simulink model "snap_adc5g_spec"  (R2019a)
settings: Solver=VariableStepDiscrete  StartTime=0.0  StopTime=10.0  RelTol=1e-3
undefined symbols (not defined in the file): pfb_coeff_gen_calc
libraries: xbsIndex_r4 x13965, casper_library_misc x80, casper_library_delays x43, xps_library x5, xbsReplacements_r4 x2, casper_library_communications x1
(part 1 of 152)
settings Model: Creator=jackh  LastModifiedBy=jackh
settings DataIOCC: ReturnWorkspaceOutputs=off
settings OptimizationCC: DefaultParameterBehavior=Inlined
settings DebuggingCC: ArithmeticOperatorsInVariantConditions=warning
settings SFSimCC: SimUseLocalCustomCode=off
settings RTWCC: RTWUseLocalCustomCode=off
settings CodeAppCC: StateflowObjectComments=on

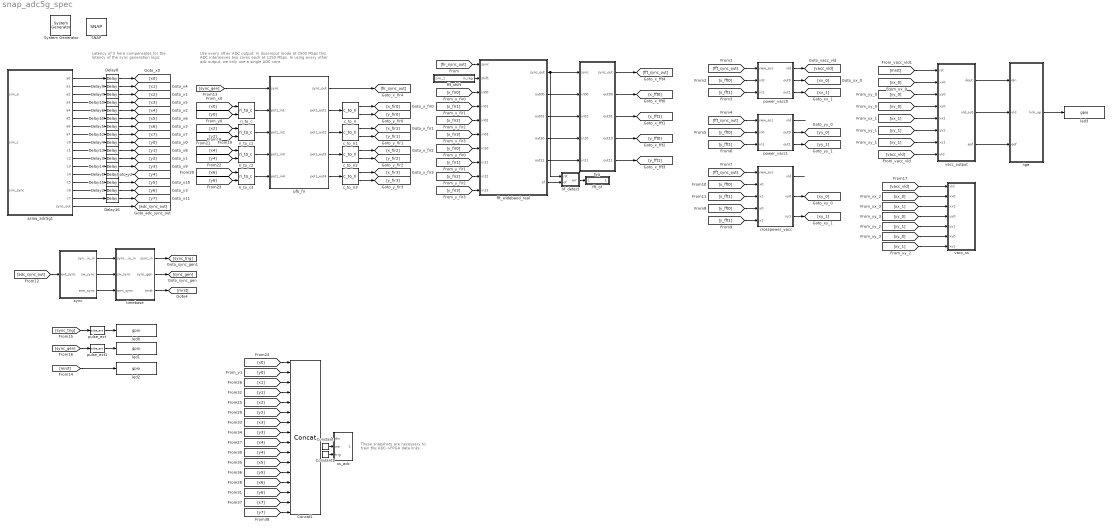
== system snap_adc5g_spec ==
  note: These snapshots are necessary
      | to train the ADC->FPGA data links.
  note: Latency of 5 here compensates
      | for the latency of the sync generation logic
  note: Use every other ADC output. In dual-input mode at 2500 MSps
      | this ADC interleaves two cores each at 1250 MSps. In using
      | every other adc output, we only use a single ADC core.
  " System Generator" : xbsIndex_r4/ System Generator  Tag=genX  xilinxfamily=kintex7  part=xc7k160t  speed=-2  package=ffg676  synthesis_tool=XST  clock_wrapper=Clock Enables  directory=/home/jackh/src/ata_snap/snap_adc5g_spec/sysgen  proj_type=Vivado  Synth_file=Vivado Synthesis Defaults  Impl_file=Vivado Implementation Defaults  testbench=off  simulink_period=1  sysclk_period=3.2  dcm_input_clock_period=10  incr_netlist=off  trim_vbits=Everywhere in SubSystem  dbl_ovrd=According to Block Masks  core_generation=According to Block Masks  run_coregen=off  deprecated_control=off  eval_field=0  block_type=sysgen
  Concat1 : xbsIndex_r4/Concat  num_inputs=16  dbl_ovrd=off  block_type=concat
  Constant : xbsIndex_r4/Constant  const=0  gui_display_data_type=Boolean  arith_type=Boolean  n_bits=16  bin_pt=14  preci_type=Single  exp_width=8  frac_width=24  explicit_period=on  period=1  equ=P=C  opselect=C  inp2=PCIN>>17  opr=+  inp1=P  carry=CIN  dbl_ovrd=off  block_type=constant
  Constant1 : xbsIndex_r4/Constant  const=0  gui_display_data_type=Boolean  arith_type=Boolean  n_bits=16  bin_pt=14  preci_type=Single  exp_width=8  frac_width=24  explicit_period=on  period=1  equ=P=C  opselect=C  inp2=PCIN>>17  opr=+  inp1=P  carry=CIN  dbl_ovrd=off  block_type=constant
  Delay{1..16} (16 alike) : xbsIndex_r4/Delay  rst=off  infoeditControl=Selection of Reset will increase slice count due to use of real FFs and instead of SRLs  en=off  latency=5  reg_retiming=off  dbl_ovrd=off  block_type=delay
      settings: block_version=11.4
  SNAP : xps_library/Platforms/SNAP  Tag=xps:xsg  hw_sys=SNAP:xc7k160t  clk_src=adc0_clk  clk_rate=1250/4  use_microblaze=on  sample_period=1  synthesis_tool=XST
      settings: SourceProductName=CASPER XPS Blockset
  asiaa_adc5g1 : Subsystem  Tag=xps:adc5g  AncestorBlock=xps_library/ADCs/asiaa_adc5g  mask(adc5g){input_mode=Two-channel -- A&C, adc_brd=ZDOK 0, demux=1:1, adc_bit_width=8, adc_clk_rate=2500, using_ctrl=on, test_ramp=off}
      mask prompts: input_mode "Input mode:"; adc_brd "ADC Board"; demux "Internal demux"; adc_bit_width "ADC Resolution (bits):"; adc_clk_rate "ADC Clock Rate (MHz):"; using_ctrl "use control"; test_ramp "start in test ramp mode"
      mask help:
      | Interface for the ASIAA 5 GSps ADC. Supports interleaving all four
      | cores using either input A or C, or interleaving two-cores each for
      | A and C. The hardware itself comes in two versions:
      |
      | DMUX 1:2 -- 4-bit samples, 4 parallel streams
      | DMUX 1:1 -- 8-bit samples, 2 parallel streams
      |
      | In either configuration this block will output 8 parallel streams
      | but the underlying interface, and the bitwidth of the samples,
      | will be different.
      mask init:
      | adc5g_init(gcb,...
      |     'input_mode', input_mode,...
      |     'demux', demux,...
      |     'adc_clk_rate', adc_clk_rate,...
      |     'adc_bit_width', adc_bit_width,...
      |     'adc_brd', adc_brd,...
      |     'using_ctrl', using_ctrl,...
      |     'test_ramp', test_ramp);
      mask TypeOptions input_mode: One-channel -- A | One-channel -- C | Two-channel -- A&C
      mask TypeOptions adc_brd: ZDOK 0 | ZDOK 1
      mask TypeOptions demux: 1:1 | 1:2
      mask Callback demux:
      | demux = get_param(gcb,'demux');
      | if(strcmp(demux,'1:1')),
      |     set_param(gcb, 'adc_bit_width', '8')
      | elseif(strcmp(demux, '1:2')),
      |     set_param(gcb, 'adc_bit_width', '4');
      | else
      | end
  c_to_ri{,1..3} (4 alike) : casper_library_misc/c_to_ri  n_bits=18  bin_pt=17
      settings: SourceProductName=CASPER DSP Blockset
  crosspower_vacc : Subsystem  mask{bw=18, nchan=2048, vacc_bw=32, vacc_bp=24}
      mask prompts: bw "Bitwidth in"; nchan "Number of channels"; vacc_bw "Vector accumulator output bitwidth"; vacc_bp "Vector accumulator output binary point"
  fft_of : Subsystem  Tag=xps:sw_reg  AncestorBlock=xps_library/Memory/software_register  mask(swreg){io_dir=To Processor, io_delay=0, init_val=0, sample_period=1, names=reg, bitwidths=1, bin_pts=0, arith_types=2, sim_port=on, show_format=on}
      mask prompts: io_dir "I/O direction"; io_delay "I/O delay"; init_val "Initial Value"; sample_period "Sample period"; names "Bitfield names [msb...lsb]"; bitwidths "Bitfield widths"; bin_pts "Bitfield binary pts"; arith_types "Bitfield types, ufix=0, fix=1, bool=2"; sim_port "Provide sim input/output?"; show_format "Print format string?"
      mask help: A 32-bit software-accessible register. Can be divided into bitfields of varying widths and types using the fields in the block mask.
      mask init:
      | swreg_init(gcb)
      settings: AttributesFormatString=1output:b = 1 bits
      mask TypeOptions io_dir: To Processor | From Processor
      mask Callback io_dir:
      | mask_enables = get_param(gcb, 'MaskEnables');
      | mask_names = get_param(gcb, 'MaskNames');
      | if strcmp(get_param(gcb, 'io_dir'), 'To Processor'),
      |     mask_enables{ismember(mask_names, 'sample_period')} = 'off';
      | else
      |     mask_enables{ismember(mask_names, 'sample_period')} = 'on';
      | end
      | set_param(gcb, 'MaskEnables', mask_enables);
      mask DialogControl ParameterTabVar0 Prompt: Setup
  fft_shift : Subsystem  Tag=xps:sw_reg  AncestorBlock=xps_library/Memory/software_register  mask(swreg){io_dir=From Processor, io_delay=0, init_val=0, sample_period=1, names=reg, bitwidths=32, bin_pts=0, arith_types=0, sim_port=on, show_format=on}
      mask prompts: io_dir "I/O direction"; io_delay "I/O delay"; init_val "Initial Value"; sample_period "Sample period"; names "Bitfield names [msb...lsb]"; bitwidths "Bitfield widths"; bin_pts "Bitfield binary pts"; arith_types "Bitfield types, ufix=0, fix=1, bool=2"; sim_port "Provide sim input/output?"; show_format "Print format string?"
      mask help: A 32-bit software-accessible register. Can be divided into bitfields of varying widths and types using the fields in the block mask.
      mask init:
      | swreg_init(gcb)
      settings: AttributesFormatString=1input:uf32.0 = 32 bits
      mask TypeOptions io_dir: To Processor | From Processor
      mask Callback io_dir:
      | mask_enables = get_param(gcb, 'MaskEnables');
      | mask_names = get_param(gcb, 'MaskNames');
      | if strcmp(get_param(gcb, 'io_dir'), 'To Processor'),
      |     mask_enables{ismember(mask_names, 'sample_period')} = 'off';
      | else
      |     mask_enables{ismember(mask_names, 'sample_period')} = 'on';
      | end
      | set_param(gcb, 'MaskEnables', mask_enables);
      mask DialogControl ParameterTabVar0 Prompt: Setup
  fft_wideband_real : Subsystem  Tag=casper:fft_wideband_real  AncestorBlock=casper_library_ffts/fft_wideband_real  mask(fft_wideband_real){n_streams=2, FFTSize=13, n_inputs=2, input_bit_width=18, bin_pt_in=17, coeff_bit_width=18, unscramble=on, async=off, floating_point=off, float_type=single, exp_width=8, frac_width=24, add_latency=1, mult_latency=2, bram_latency=3, conv_latency=1, input_latency=0, biplex_direct_latency=0, add_pipe_latency=0, mult_pipe_latency=0, quantization=Round  (unbiased: Even Values), overflow=Wrap, delays_bit_limit=8, coeffs_bit_limit=9, coeff_sharing=on, coeff_decimation=on, coeff_generation=off, cal_bits=1, n_bits_rotation=25, mult_spec=2, max_fanout=4, bitgrowth=off, max_bits=19, hardcode_shifts=off, shift_schedule=[], dsp48_adders=off}
      mask prompts: n_streams "Number simultaneous streams"; FFTSize "Size of FFT: (2^? pts)"; n_inputs "Number of Simultaneous Inputs: (2^?)"; input_bit_width "Input Bit Width"; bin_pt_in "Input binary point"; coeff_bit_width "Coefficient Bit Width"; unscramble "Unscramble output (ie, put channels in canonical order)"; async "Asynchronous operation"; floating_point "floating point"; float_type "float type"; exp_width "exponent width"; frac_width "fraction width"; add_latency "Add Latency"; mult_latency "Mult Latency"; bram_latency "BRAM Latency"; conv_latency "Convert Latency"; input_latency "Input Latency"; biplex_direct_latency "Latency between biplexes and fft_direct"; add_pipe_latency "Add Interface Pipeline Latency"; mult_pipe_latency "CMult Pipeline Latency"; quantization "Quantization Behavior"; overflow "Overflow Behavior"; delays_bit_limit "Number bits above which to store stage's delays in BRAM (2^? bits)"; coeffs_bit_limit "Number bits above which to store stage's coefficients in BRAM (2^? bits)"; coeff_sharing "BRAM sharing in coeff storage"; coeff_decimation "Store a fraction of coeff factors where useful"; coeff_generation "Generate coeffs with multipliers where useful"; cal_bits "Number calibration locations when generating coeffs (2^?)"; n_bits_rotation "Feedback rotation vector resolution"; mult_spec "Multiplier impl. (0=core, 1=embedded, 2=behavioural) (left=1st stage, or just one value)"; max_fanout "Maximum fanout"; bitgrowth "Bitgrowth instead of shifting"; max_bits "Max bits to grow to"; hardcode_shifts "Hardcode shift schedule"; shift_schedule "Shift schedule"; dsp48_adders "DSP48 adders in butterfly"
      mask help: A real-sampled wideband FFT.
      mask init:
      | fft_wideband_real_init(gcb, ...
      |     'n_streams', n_streams, ...
      |     'FFTSize', FFTSize, ...
      |     'n_inputs', n_inputs, ...
      |     'input_bit_width', input_bit_width, ...
      |     'bin_pt_in', bin_pt_in, ...
      |     'coeff_bit_width', coeff_bit_width, ...
      |     'floating_point', floating_point, ...
      |     'float_type', float_type, ...
      |     'exp_width', exp_width, ...
      |     'frac_width', frac_width, ...
      |     'unscramble', unscramble, ...
      |     'async', async, ...
      |     'add_latency', add_latency, ...
      |     'mult_latency', mult_latency, ...
      |     'bram_latency', bram_latency, ...
      |     'conv_latency', conv_latency, ...
      |     'input_latency', input_latency, ...
      |     'add_pipe_latency', add_pipe_latency, ...
      |     'mult_pipe_latency', mult_pipe_latency, ...
      |     'biplex_direct_latency', biplex_direct_latency, ...
      |     'quantization', quantization, ...
      |     'overflow', overflow, ...
      |     'delays_bit_limit', delays_bit_limit, ...
      |     'coeffs_bit_limit', coeffs_bit_limit, ...
      |     'coeff_sharing', coeff_sharing, ...
      |     'coeff_decimation', coeff_decimation, ...
      |     'coeff_generation', coeff_generation, ...
      |     'cal_bits', cal_bits, ...
      |     'n_bits_rotation', n_bits_rotation, ...
      |     'max_fanout', max_fanout, ...   
      |     'mult_spec', mult_spec, ...
      |     'bitgrowth', bitgrowth, ...
      |     'max_bits', max_bits, ...
      |     'hardcode_shifts', hardcode_shifts, ...
      |     'shift_schedule', shift_schedule, ...
      |     'dsp48_adders', dsp48_adders);
      settings: AttributesFormatString=|
      | 13 stages
      | (18,18)
      | Round  (unbiased: Even Values)
      | Wrap
      mask Help: eval('xlWeb(''http://casper.berkeley.edu/wiki/Fft_wideband_real'')')
      mask Callback floating_point:
      | onoff = get_param(gcb, 'floating_point');
      | if strcmp(onoff,'on')
      |     enable_fixpt = 'off'
      |     set_param_state(gcb, 'float_type', 'on')
      | 
      |     f_type = get_param(gcb, 'float_type')
      |     if strcmp(f_type,'custom')
      |         set_param_state(gcb, 'exp_width', 'on')
      |         set_param_state(gcb, 'frac_width', 'on')
      |     else
      |         set_param_state(gcb, 'exp_width', 'off')
      |         set_param_state(gcb, 'frac_width', 'off')
      |     end
      | 
      | 
      | else
      |     enable_fixpt = 'on'
      |     set_param_state(gcb, 'float_type', 'off')
      |     set_param_state(gcb, 'exp_width', 'off')
      |     set_param_state(gcb, 'frac_width', 'off')
      | end
      | 
      | set_param_state(gcb, 'input_bit_width', enable_fixpt)
      | set_param_state(gcb, 'bin_pt_in', enable_fixpt)
      | set_param_state(gcb, 'coeff_bit_width', enable_fixpt)
      mask TypeOptions float_type: single | custom
      mask Callback float_type:
      | f_type = get_param(gcb, 'float_type')
      | if strcmp(f_type,'custom')
      |     set_param_state(gcb, 'exp_width', 'on')
      |     set_param_state(gcb, 'frac_width', 'on')
      | else
      |     set_param_state(gcb, 'exp_width', 'off')
      |     set_param_state(gcb, 'frac_width', 'off')
      | end
      mask TypeOptions quantization: Truncate | Round  (unbiased: +/- Inf) | Round  (unbiased: Even Values)
      mask TypeOptions overflow: Wrap | Saturate | Error
      mask Callback hardcode_shifts:
      | hardcode_shifts = get_param(gcb, 'hardcode_shifts');
      | set_param_state(gcb, 'shift_schedule', hardcode_shifts);
      mask Callback dsp48_adders: fft_callback_dsp48_adders(gcb);
      mask DialogControl ParameterTabVar0 Prompt: Basic
      mask DialogControl ParameterTabVar01 Prompt: Latency
      mask DialogControl ParameterTabVar012 Prompt: Implementation
  led0 : xps_library/IO/gpio  Tag=xps:gpio  io_group_params_forwarded=on  io_group=ROACH:led  io_group_real=led  io_group_custom=0  io_dir=out  arith_type=Boolean  bitwidth=1  bin_pt=0  bit_index=0  sample_period=1  use_single_ended=off  use_ddr=off  reg_iob=on  reg_clk_phase=0  termination=None
      settings: SourceProductName=CASPER XPS Blockset
  led1 : xps_library/IO/gpio  Tag=xps:gpio  io_group_params_forwarded=on  io_group=ROACH:led  io_group_real=led  io_group_custom=0  io_dir=out  arith_type=Boolean  bitwidth=1  bin_pt=0  bit_index=1  sample_period=1  use_single_ended=off  use_ddr=off  reg_iob=on  reg_clk_phase=0  termination=None
      settings: SourceProductName=CASPER XPS Blockset
  led2 : xps_library/IO/gpio  Tag=xps:gpio  io_group_params_forwarded=on  io_group=ROACH:led  io_group_real=led  io_group_custom=0  io_dir=out  arith_type=Boolean  bitwidth=1  bin_pt=0  bit_index=2  sample_period=1  use_single_ended=off  use_ddr=off  reg_iob=on  reg_clk_phase=0  termination=None
      settings: SourceProductName=CASPER XPS Blockset
  led3 : xps_library/IO/gpio  Tag=xps:gpio  io_group_params_forwarded=on  io_group=ROACH:led  io_group_real=led  io_group_custom=0  io_dir=out  arith_type=Boolean  bitwidth=1  bin_pt=0  bit_index=3  sample_period=1  use_single_ended=off  use_ddr=off  reg_iob=on  reg_clk_phase=0  termination=None
      settings: SourceProductName=CASPER XPS Blockset
  of_detect : Subsystem
  pfb_fir : Subsystem  Tag=casper:pfb_fir  AncestorBlock=casper_library_pfbs/pfb_fir  mask(pfb_fir){PFBSize=13, TotalTaps=8, WindowType=hamming, n_inputs=2, MakeBiplex=off, BitWidthIn=8, BitWidthOut=18, CoeffBitWidth=18, CoeffDistMem=off, add_latency=1, mult_latency=2, bram_latency=3, fan_latency=1, quantization=Round  (unbiased: Even Values), fwidth=1, mult_spec=2, coeffs_share=on}
      mask prompts: PFBSize "Size of PFB: (2^? pnts)"; TotalTaps "Total Number of Taps:"; WindowType "Windowing Function:"; n_inputs "Number of Simultaneous Inputs: (2^?)"; MakeBiplex "Make Biplex?"; BitWidthIn "Input Bitwidth:"; BitWidthOut "Output Bitwidth:"; CoeffBitWidth "Coefficient Bitwidth:"; CoeffDistMem "Use Distributed Memory for Coeffs"; add_latency "Add Latency"; mult_latency "Mult Latency"; bram_latency "BRAM Latency"; fan_latency "Fanout Latency"; quantization "Quantization Behavior"; fwidth "Bin Width Scaling (normal=1)"; mult_spec "Multiplier specification (0=core, 1=embedded, 2=behavioural) (left=1st tap, or just one value)"; coeffs_share "Share coefficients between polarisations (use less BRAM)?"
      mask init:
      | pfb_fir_init(gcb, ...
      |     'PFBSize', PFBSize, ...
      |     'TotalTaps', TotalTaps, ...
      |     'WindowType', WindowType, ...
      |     'n_inputs', n_inputs, ...
      |     'MakeBiplex', MakeBiplex, ...
      |     'BitWidthIn', BitWidthIn, ...
      |     'BitWidthOut', BitWidthOut, ...
      |     'CoeffBitWidth', CoeffBitWidth, ...
      |     'CoeffDistMem', CoeffDistMem, ...
      |     'add_latency', add_latency, ...
      |     'mult_latency', mult_latency, ...
      |     'bram_latency', bram_latency, ...
      |     'fan_latency', fan_latency, ...
      |     'quantization', quantization, ...
      |     'fwidth', fwidth, ...
      |     'mult_spec', mult_spec, ...
      |     'coeffs_share', coeffs_share);
      settings: AttributesFormatString=|
      | taps=8, add_latency=1
      | max scale 0.823
      mask Help: eval('xlWeb(''http://casper.berkeley.edu/wiki/Pfb_fir'')')
      mask Callback TotalTaps:
      | %num_taps = eval(get_param(gcb, 'TotalTaps'));
      | %old_vec = eval(get_param(gcb, 'mult_spec'));
      | 
      | %vec = 2.*ones(1,num_taps);
      | %old_size = length(old_vec);
      | 
      | %if(old_size <= num_taps),
      | %   new_size = old_size;
      | %else,
      | %    new_size = num_taps;
      | %end
      | 
      | %for n = 1:new_size, vec(n) = old_vec(n); end
      | %set_param(gcb, 'mult_spec', mat2str(vec));
      mask TypeOptions WindowType: bartlett | barthannwin | blackman | blackmanharris | bohamwin | chebwin | flattopwin | gausswin | hamming | hann | kaiser | nuttallwin | parzenwin | rectwin | tukeywin | triang | userwindow
      mask TypeOptions quantization: Truncate | Round  (unbiased: +/- Inf) | Round  (unbiased: Even Values)
      mask Callback fwidth:
      | %num_taps = eval(get_param(gcb, 'TotalTaps'));
      | %old_vec = eval(get_param(gcb, 'mult_spec'));
      | 
      | %vec = 2.*ones(1,num_taps);
      | %old_size = length(old_vec);
      | 
      | %if(old_size <= num_taps),
      | %    new_size = old_size;
      | %else,
      | %    new_size = num_taps;
      | %end
      | 
      | %for n = 1:new_size, vec(n) = old_vec(n); end
      | %set_param(gcb, 'mult_spec', mat2str(vec));
      mask Callback mult_spec:
      | %num_taps = eval(get_param(gcb, 'TotalTaps'));
      | %old_vec = eval(get_param(gcb, 'mult_spec'));
      | 
      | %vec = 2.*ones(1,num_taps);
      | %old_size = length(old_vec);
      | 
      | %if(old_size <= num_taps),
      | %    new_size = old_size;
      | %else,
      | %    new_size = num_taps;
      | %end
      | 
      | %for n = 1:new_size, vec(n) = old_vec(n); end
      | %set_param(gcb, 'mult_spec', mat2str(vec));
  power_vacc0 : Subsystem  mask{bw=18, nchan=2048, vacc_bw=32, vacc_bp=24}
      mask prompts: bw "Bitwidth in"; nchan "Number of channels"; vacc_bw "Vector accumulator output bitwidth"; vacc_bp "Vector accumulator output binary point"
  power_vacc1 : Subsystem  mask{bw=18, nchan=2048, vacc_bw=32, vacc_bp=24}
      mask prompts: bw "Bitwidth in"; nchan "Number of channels"; vacc_bw "Vector accumulator output bitwidth"; vacc_bp "Vector accumulator output binary point"
  pulse_ext : casper_library_misc/pulse_ext  pulse_len=2^25
      settings: SourceProductName=CASPER DSP Blockset
  pulse_ext1 : casper_library_misc/pulse_ext  pulse_len=2^25
      settings: SourceProductName=CASPER DSP Blockset
  ri_to_c{,1..3} (4 alike) : casper_library_misc/ri_to_c
      settings: SourceProductName=CASPER DSP Blockset
  ss_adc : Subsystem  Tag=casper:snapshot  AncestorBlock=casper_library_scopes/snapshot  mask(snapshot){storage=bram, dram_dimm=1, dram_clock=200, nsamples=10, data_width=128, offset=off, circap=off, value=off, ext_arm=off, ext_circ=off, provide_outputs=on, use_dsp48=off}
      mask prompts: storage "Storage medium"; dram_dimm "DRAM dimm"; dram_clock "DRAM clock rate"; nsamples "Number of Samples (2^?)"; data_width "Data width"; offset "Start delay support"; circap "Circular capture support"; value "Extra value capture support"; ext_arm "External arm support"; ext_circ "External circular capture support"; provide_outputs "Provide outputs"; use_dsp48 "Use DSP48s to implement counters"
      mask help:
      | Standard snap block, but with the following optional extras;
      |  1) Optionally delay the fabric trigger by a user-specified number of valids.
      |  2) Capture continuously after a trigger until a stop pulse is received. Data is captured into BRAM continuously, with old data being overwritten until a stop command is received. Then stop capturing when memory is filled. This enables you to get some data before and some data after the stop pulse. Use the 'tr_en_cnt' register to determine where you are in your vector. 'Addr' register's MSb now indicates 'busy capturing'.
      |  3) Optionally capture a value on an input port to a register at the same time as the first data sample.
      |  4) Implement counters using DSP48Es to save resources.
      mask init:
      | snapshot_init(gcb, ...
      |     'storage', storage, ...
      |     'dram_dimm', dram_dimm, ...
      |     'dram_clock', dram_clock, ...
      |     'nsamples', nsamples, ...
      |     'data_width', data_width, ...
      |     'offset', offset, ...
      |     'circap', circap, ...
      |     'value', value, ...
      |     'ext_arm', ext_arm, ...
      |     'ext_circ', ext_circ, ...
      |     'provide_outputs', 'off', ...
      |     'use_dsp48', use_dsp48);
      settings: AttributesFormatString=|
      | 128 wide, 1024 deep
      | debugID: 76998629
      mask TypeOptions storage: bram | dram
      mask Callback storage: snapshot_callback();
      mask TypeOptions dram_dimm: 1 | 2 | 3 | 4
      mask TypeOptions dram_clock: 200 | 250 | 266 | 300 | 333
      mask TypeOptions data_width: 8 | 16 | 32 | 64 | 128
  sync : Subsystem
  tge : Subsystem
  timebase : Subsystem
  tvg : Subsystem
  vacc_output : Subsystem
  vacc_ss : Subsystem
  wires:
  [sync_gen] -> pfb_fir/1(sync)
  ri_to_c/1 -> pfb_fir/2(pol1_in1)
  ri_to_c2/1 -> pfb_fir/4(pol1_in3)
  ri_to_c3/1 -> pfb_fir/5(pol1_in4)
  ri_to_c1/1 -> pfb_fir/3(pol1_in2)
  [x0] -> ri_to_c/1
  [x2] -> ri_to_c1/1
  [x4] -> ri_to_c2/1
  [x6] -> ri_to_c3/1
  [y0] -> ri_to_c/2
  [y2] -> ri_to_c1/2
  [y4] -> ri_to_c2/2
  [y6] -> ri_to_c3/2
  pfb_fir/2(pol1_out1) -> c_to_ri/1
  pfb_fir/3(pol1_out2) -> c_to_ri1/1
  pfb_fir/4(pol1_out3) -> c_to_ri2/1
  pfb_fir/5(pol1_out4) -> c_to_ri3/1
  c_to_ri/1 -> [x_fir0]
  c_to_ri2/2 -> [y_fir2]
  c_to_ri/2 -> [y_fir0]
  c_to_ri1/1 -> [x_fir1]
  c_to_ri1/2 -> [y_fir1]
  c_to_ri2/1 -> [x_fir2]
  c_to_ri3/1 -> [x_fir3]
  c_to_ri3/2 -> [y_fir3]
  [x_fir0] -> fft_wideband_real/3(in00)
  [y_fir0] -> fft_wideband_real/7(in10)
  [x_fir1] -> fft_wideband_real/4(in01)
  [y_fir1] -> fft_wideband_real/8(in11)
  [x_fir2] -> fft_wideband_real/5(in02)
  [y_fir2] -> fft_wideband_real/9(in12)
  [x_fir3] -> fft_wideband_real/6(in03)
  [y_fir3] -> fft_wideband_real/10(in13)
  pfb_fir/1(sync_out) -> [fir_sync_out]
  [fir_sync_out] -> fft_wideband_real/1(sync)
  fft_shift/1(in_reg) -> fft_wideband_real/2(shift)
  fft_wideband_real/1(sync_out) -> tvg/1(sync), of_detect/1(rst)
  sync/1(sync_gpio_in) -> timebase/1(sync_gpio_in)
  sync/2(sw_sync) -> timebase/2(sw_sync)
  sync/3(arm_sync) -> timebase/3(arm_sync)
  timebase/2(sync_gen) -> [sync_gen]
  timebase/1(sync_in) -> [sync_trig]
  timebase/3(mrst) -> [mrst]
  [adc_sync_out] -> sync/1(ext_sync)
  [mrst] -> led2/1
  pulse_ext/1 -> led0/1
  pulse_ext1/1 -> led1/1
  [sync_trig] -> pulse_ext/1
  [sync_gen] -> pulse_ext1/1
  Delay2/1 -> [y6]
  Delay1/1 -> [y4]
  Delay3/1 -> [y2]
  Delay4/1 -> [y0]
  Delay5/1 -> [x6]
  Delay6/1 -> [x4]
  Delay7/1 -> [x2]
  Delay8/1 -> [x0]
  fft_wideband_real/6(of) -> of_detect/2(of)
  of_detect/1(err) -> fft_of/1(out_reg)
  Concat1/1 -> ss_adc/1(din)
  Constant/1 -> ss_adc/2(we)
  Constant1/1 -> ss_adc/3(trig)
  tvg/1(sync_out) -> [fft_sync_out]
  tvg/4(out10) -> [y_fft0]
  tvg/3(out01) -> [x_fft1]
  tvg/5(out11) -> [y_fft1]
  tvg/2(out00) -> [x_fft0]
  fft_wideband_real/2(out00) -> tvg/2(in00)
  fft_wideband_real/3(out01) -> tvg/3(in01)
  fft_wideband_real/4(out10) -> tvg/4(in10)
  fft_wideband_real/5(out11) -> tvg/5(in11)
  Delay9/1 -> [x1]
  Delay10/1 -> [x3]
  Delay11/1 -> [x5]
  Delay12/1 -> [x7]
  Delay13/1 -> [y1]
  Delay14/1 -> [y3]
  Delay15/1 -> [y5]
  Delay16/1 -> [y7]
  [x0] -> Concat1/1
  [y0] -> Concat1/2
  [x2] -> Concat1/5
  [y2] -> Concat1/6
  [x4] -> Concat1/9
  [y4] -> Concat1/10
  [x6] -> Concat1/13
  [x1] -> Concat1/3
  [y1] -> Concat1/4
  [x3] -> Concat1/7
  [y3] -> Concat1/8
  [x5] -> Concat1/11
  [y5] -> Concat1/12
  [y6] -> Concat1/14
  [x7] -> Concat1/15
  [y7] -> Concat1/16
  [fft_sync_out] -> power_vacc0/1(new_acc)
  [x_fft0] -> power_vacc0/2(in0)
  [x_fft1] -> power_vacc0/3(in1)
  [fft_sync_out] -> power_vacc1/1(new_acc)
  [y_fft0] -> power_vacc1/2(in0)
  [y_fft1] -> power_vacc1/3(in1)
  [fft_sync_out] -> crosspower_vacc/1(new_acc)
  [x_fft0] -> crosspower_vacc/2(x0)
  [x_fft1] -> crosspower_vacc/3(x1)
  [y_fft1] -> crosspower_vacc/5(y1)
  [y_fft0] -> crosspower_vacc/4(y0)
  power_vacc1/1(vld) -> ?
  power_vacc0/2(out0) -> [xx_0]
  power_vacc0/3(out1) -> [xx_1]
  power_vacc1/2(out0) -> [yy_0]
  power_vacc1/3(out1) -> [yy_1]
  crosspower_vacc/1(vld) -> ?
  crosspower_vacc/2(xy0) -> [xy_0]
  crosspower_vacc/3(xy1) -> [xy_1]
  power_vacc0/1(vld) -> [vacc_vld]
  [mrst] -> vacc_output/1(rst)
  [xx_0] -> vacc_output/2(xx0)
  [yy_0] -> vacc_output/3(yy0)
  [xy_0] -> vacc_output/4(xy0)
  [xx_1] -> vacc_output/5(xx1)
  [yy_1] -> vacc_output/6(yy1)
  [xy_1] -> vacc_output/7(xy1)
  [vacc_vld] -> vacc_output/8(vld)
  [xx_0] -> vacc_ss/2(xx0)
  [xx_1] -> vacc_ss/3(xx1)
  [yy_0] -> vacc_ss/4(yy0)
  [yy_1] -> vacc_ss/5(yy1)
  [xy_0] -> vacc_ss/6(xy0)
  [xy_1] -> vacc_ss/7(xy1)
  [vacc_vld] -> vacc_ss/1(vld)
  vacc_output/1(dout) -> tge/1(din)
  vacc_output/2(vld_out) -> tge/2(vld)
  vacc_output/3(eof) -> tge/3(eof)
  tge/1(link_up) -> led3/1
  asiaa_adc5g1/1(a0) -> Delay8/1
  asiaa_adc5g1/2(a1) -> Delay9/1
  asiaa_adc5g1/3(a2) -> Delay7/1
  asiaa_adc5g1/4(a3) -> Delay10/1
  asiaa_adc5g1/5(a4) -> Delay6/1
  asiaa_adc5g1/6(a5) -> Delay11/1
  asiaa_adc5g1/7(a6) -> Delay5/1
  asiaa_adc5g1/8(a7) -> Delay12/1
  asiaa_adc5g1/9(c0) -> Delay4/1
  asiaa_adc5g1/10(c1) -> Delay13/1
  asiaa_adc5g1/11(c2) -> Delay3/1
  asiaa_adc5g1/12(c3) -> Delay14/1
  asiaa_adc5g1/13(c4) -> Delay1/1
  asiaa_adc5g1/14(c5) -> Delay15/1
  asiaa_adc5g1/15(c6) -> Delay2/1
  asiaa_adc5g1/16(c7) -> Delay16/1
  asiaa_adc5g1/17(sync_out) -> [adc_sync_out]

== system snap_adc5g_spec/asiaa_adc5g1 ==
  sim_a : Inport
  sim_c : Inport  Port=2
  sim_sync : Inport  Port=3
  bias_a : Bias  Bias=128  SaturateOnIntegerOverflow=on
  bias_c : Bias  Bias=128  SaturateOnIntegerOverflow=on
  gain_a : Gain  Gain=128  SaturateOnIntegerOverflow=on  OutDataTypeStr=Inherit: Same as input  ParamDataTypeStr=Inherit: Same as input
  gain_c : Gain  Gain=128  SaturateOnIntegerOverflow=on  OutDataTypeStr=Inherit: Same as input  ParamDataTypeStr=Inherit: Same as input
  snap_adc5g_spec_asiaa_adc5g1_sync : xbsIndex_r4/Gateway In  gui_display_data_type=Fixed-point  arith_type=Boolean  n_bits=16  bin_pt=14  preci_type=Single  exp_width=8  frac_width=24  rows=1  columns=1  quantization="Round  (unbiased: +/- Inf)"  overflow=Saturate  period=1  UseAsADC=off  ADCChannel='1'  interface=None  automatic_assignment=on  address_offset=hex2dec('00')  intf_name=''  intf_description=''  default_value=0  timing_constraint=None  locs_specified=off  LOCs={}  io_standard={}  inherit_from_input=off  hdl_port=on  dbl_ovrd=off  block_type=gatewayin
  snap_adc5g_spec_asiaa_adc5g1_user_data_i{0..7} (8 alike) : xbsIndex_r4/Gateway In  gui_display_data_type=Fixed-point  arith_type=Unsigned  n_bits=8  bin_pt=0  preci_type=Single  exp_width=8  frac_width=24  rows=1  columns=1  quantization=Truncate  overflow=Wrap  period=1  UseAsADC=off  ADCChannel='1'  interface=None  automatic_assignment=on  address_offset=hex2dec('00')  intf_name=''  intf_description=''  default_value=0  timing_constraint=None  locs_specified=off  LOCs={}  io_standard={}  inherit_from_input=off  hdl_port=on  dbl_ovrd=off  block_type=gatewayin
  snap_adc5g_spec_asiaa_adc5g1_user_data_q{0..7} (8 alike) : xbsIndex_r4/Gateway In  gui_display_data_type=Fixed-point  arith_type=Unsigned  n_bits=8  bin_pt=0  preci_type=Single  exp_width=8  frac_width=24  rows=1  columns=1  quantization=Truncate  overflow=Wrap  period=1  UseAsADC=off  ADCChannel='1'  interface=None  automatic_assignment=on  address_offset=hex2dec('00')  intf_name=''  intf_description=''  default_value=0  timing_constraint=None  locs_specified=off  LOCs={}  io_standard={}  inherit_from_input=off  hdl_port=on  dbl_ovrd=off  block_type=gatewayin
  a0 : Outport
  a1 : Outport  Port=2
  a2 : Outport  Port=3
  a3 : Outport  Port=4
  a4 : Outport  Port=5
  a5 : Outport  Port=6
  a6 : Outport  Port=7
  a7 : Outport  Port=8
  c0 : Outport  Port=9
  c1 : Outport  Port=10
  c2 : Outport  Port=11
  c3 : Outport  Port=12
  c4 : Outport  Port=13
  c5 : Outport  Port=14
  c6 : Outport  Port=15
  c7 : Outport  Port=16
  sync_out : Outport  Port=17
  wires:
  sim_a/1 -> gain_a/1
  gain_a/1 -> bias_a/1
  bias_a/1 -> snap_adc5g_spec_asiaa_adc5g1_user_data_i0/1, snap_adc5g_spec_asiaa_adc5g1_user_data_i1/1, snap_adc5g_spec_asiaa_adc5g1_user_data_i2/1, snap_adc5g_spec_asiaa_adc5g1_user_data_i3/1, snap_adc5g_spec_asiaa_adc5g1_user_data_i4/1, snap_adc5g_spec_asiaa_adc5g1_user_data_i5/1, snap_adc5g_spec_asiaa_adc5g1_user_data_i6/1, snap_adc5g_spec_asiaa_adc5g1_user_data_i7/1
  snap_adc5g_spec_asiaa_adc5g1_user_data_i0/1 -> a0/1
  snap_adc5g_spec_asiaa_adc5g1_user_data_i1/1 -> a1/1
  snap_adc5g_spec_asiaa_adc5g1_user_data_i2/1 -> a2/1
  snap_adc5g_spec_asiaa_adc5g1_user_data_i3/1 -> a3/1
  snap_adc5g_spec_asiaa_adc5g1_user_data_i4/1 -> a4/1
  snap_adc5g_spec_asiaa_adc5g1_user_data_i5/1 -> a5/1
  snap_adc5g_spec_asiaa_adc5g1_user_data_i6/1 -> a6/1
  snap_adc5g_spec_asiaa_adc5g1_user_data_i7/1 -> a7/1
  sim_c/1 -> gain_c/1
  gain_c/1 -> bias_c/1
  bias_c/1 -> snap_adc5g_spec_asiaa_adc5g1_user_data_q0/1, snap_adc5g_spec_asiaa_adc5g1_user_data_q1/1, snap_adc5g_spec_asiaa_adc5g1_user_data_q2/1, snap_adc5g_spec_asiaa_adc5g1_user_data_q3/1, snap_adc5g_spec_asiaa_adc5g1_user_data_q4/1, snap_adc5g_spec_asiaa_adc5g1_user_data_q5/1, snap_adc5g_spec_asiaa_adc5g1_user_data_q6/1, snap_adc5g_spec_asiaa_adc5g1_user_data_q7/1
  snap_adc5g_spec_asiaa_adc5g1_user_data_q0/1 -> c0/1
  snap_adc5g_spec_asiaa_adc5g1_user_data_q1/1 -> c1/1
  snap_adc5g_spec_asiaa_adc5g1_user_data_q2/1 -> c2/1
  snap_adc5g_spec_asiaa_adc5g1_user_data_q3/1 -> c3/1
  snap_adc5g_spec_asiaa_adc5g1_user_data_q4/1 -> c4/1
  snap_adc5g_spec_asiaa_adc5g1_user_data_q5/1 -> c5/1
  snap_adc5g_spec_asiaa_adc5g1_user_data_q6/1 -> c6/1
  snap_adc5g_spec_asiaa_adc5g1_user_data_q7/1 -> c7/1
  sim_sync/1 -> snap_adc5g_spec_asiaa_adc5g1_sync/1
  snap_adc5g_spec_asiaa_adc5g1_sync/1 -> sync_out/1

== system snap_adc5g_spec/crosspower_vacc ==
  new_acc : Inport
  x0 : Inport  Port=2
  x1 : Inport  Port=3
  y0 : Inport  Port=4
  y1 : Inport  Port=5
  Convert{1..4} (4 alike) : xbsIndex_r4/Convert  gui_display_data_type=Fixed-point  arith_type="Signed  (2's comp)"  n_bits=25  bin_pt=24  float_type=Single  exp_bits=8  fraction_bits=24  quantization="Round  (unbiased: Even Values)"  overflow=Saturate  en=off  latency=2  pipeline=off  dbl_ovrd=off  block_type=convert
  Counter : xbsIndex_r4/Counter  cnt_type=Free Running  cnt_to=Inf  operation=Up  start_count=0  cnt_by_val=1  arith_type=Unsigned  n_bits=32  bin_pt=0  load_pin=off  rst=on  en=on  explicit_period=on  period=1  use_behavioral_HDL=off  implementation=Fabric  dbl_ovrd=off  block_type=counter
  Delay : xbsIndex_r4/Delay  rst=off  infoeditControl=Selection of Reset will increase slice count due to use of real FFs and instead of SRLs  en=off  latency=4  reg_retiming=off  dbl_ovrd=off  block_type=delay
  Delay1 : xbsIndex_r4/Delay  rst=off  infoeditControl=Selection of Reset will increase slice count due to use of real FFs and instead of SRLs  en=off  latency=2  reg_retiming=off  dbl_ovrd=off  block_type=delay
  Logical : xbsIndex_r4/Logical  logical_function=OR  inputs=4  en=off  latency=1  precision=Full  arith_type=Unsigned  n_bits=16  bin_pt=0  align_bp=on  dbl_ovrd=off  block_type=logical
  Register : xbsIndex_r4/Register  init=0  rst=off  en=on  dbl_ovrd=off  block_type=register
  c_to_ri : casper_library_misc/c_to_ri  n_bits=bw+bw+1  bin_pt=bw-1 + bw-1
      settings: AttributesFormatString=37_34 r/i  SourceProductName=CASPER DSP Blockset
  c_to_ri1 : casper_library_misc/c_to_ri  n_bits=bw+bw+1  bin_pt=bw-1 + bw-1
      settings: AttributesFormatString=37_34 r/i  SourceProductName=CASPER DSP Blockset
  cmult : Subsystem  AncestorBlock=casper_library_multipliers/cmult  mask(cmult){n_bits_a=bw, bin_pt_a=bw-1, n_bits_b=bw, bin_pt_b=bw-1, n_bits_ab=bw+bw+1, bin_pt_ab=bw-1 + bw-1, quantization=Truncate, overflow=Wrap, conjugated=on, async=off, pipelined_enable=off, floating_point=off, float_type=single, exp_width=8, frac_width=24, in_latency=0, mult_latency=3, add_latency=1, conv_latency=0, pipeline_cmult_en=off, pipeline_latency=0, multiplier_implementation=behavioral HDL}
      mask prompts: n_bits_a "Number of Bits 'a'"; bin_pt_a "Binary Point 'a'"; n_bits_b "Number of Bits 'b'"; bin_pt_b "Binary Point 'b'"; n_bits_ab "Number of Bits 'ab'"; bin_pt_ab "Binary Point 'ab'"; conjugated "Conjugate"; async "asynchronous operation"; pipelined_enable "enable pipeline"; floating_point "floating point"; float_type "float type"; exp_width "exponent width"; frac_width "fraction width"; in_latency "Input latency"; mult_latency "Multiplier Latency"; add_latency "Adder Latency"; conv_latency "Convert latency"; pipeline_cmult_en "Pipeline cmult enable"; pipeline_latency "Pipeline latency"; multiplier_implementation "Multiplier implementation"
      mask help:
      | Multiplies two complex numbers using 4 multipliers and 2 adders.
      | Conjugation is optional.
      mask init:
      | cmult_init(gcb, ...
      |     'n_bits_a',n_bits_a, ...
      |     'bin_pt_a',bin_pt_a, ...
      |     'n_bits_b',n_bits_b, ...
      |     'bin_pt_b',bin_pt_b, ...
      |     'n_bits_ab',n_bits_ab, ...
      |     'bin_pt_ab',bin_pt_ab, ...
      |     'quantization',quantization, ...
      |     'floating_point', floating_point, ...
      |     'float_type', float_type, ...
      |     'exp_width', exp_width, ...
      |     'frac_width', frac_width, ...    
      |     'overflow', overflow, ...
      |     'in_latency', in_latency, ...
      |     'mult_latency', mult_latency, ...
      |     'add_latency', add_latency, ...
      |     'conv_latency', conv_latency, ...
      |     'conjugated', conjugated, ...
      |     'pipeline_cmult_en', pipeline_cmult_en, ...
      |     'pipeline_latency', pipeline_latency, ...
      |     'multiplier_implementation', multiplier_implementation, ...
      |     'async', async, ...
      |     'pipelined_enable', pipelined_enable);
      settings: AttributesFormatString=|
      | 18_17 * 18_17 ==> 37_34
      | Truncate, Wrap
      | Latency=0
      mask TypeOptions quantization: Truncate | Round  (unbiased: +/- Inf) | Round  (unbiased: Even Values)
      mask TypeOptions overflow: Wrap | Saturate | Flag as error
      mask Callback floating_point:
      | onoff = get_param(gcb, 'floating_point');
      | if strcmp(onoff,'on')
      |     enable_fixpt = 'off'
      |     set_param_state(gcb, 'float_type', 'on')
      | 
      |     f_type = get_param(gcb, 'float_type')
      |     if strcmp(f_type,'custom')
      |         set_param_state(gcb, 'exp_width', 'on')
      |         set_param_state(gcb, 'frac_width', 'on')
      |     else
      |         set_param_state(gcb, 'exp_width', 'off')
      |         set_param_state(gcb, 'frac_width', 'off')
      |     end
      | 
      | 
      | else
      |     enable_fixpt = 'on'
      |     set_param_state(gcb, 'float_type', 'off')
      |     set_param_state(gcb, 'exp_width', 'off')
      |     set_param_state(gcb, 'frac_width', 'off')
      | end
      | 
      | 
      | set_param_state(gcb, 'n_bits_a', enable_fixpt)
      | set_param_state(gcb, 'bin_pt_a', enable_fixpt)
      | set_param_state(gcb, 'n_bits_b', enable_fixpt)
      | set_param_state(gcb, 'bin_pt_b', enable_fixpt)
      | set_param_state(gcb, 'n_bits_ab', enable_fixpt)
      | set_param_state(gcb, 'bin_pt_ab', enable_fixpt)
      mask TypeOptions float_type: single | custom
      mask Callback float_type:
      | f_type = get_param(gcb, 'float_type')
      | if strcmp(f_type,'custom')
      |     set_param_state(gcb, 'exp_width', 'on')
      |     set_param_state(gcb, 'frac_width', 'on')
      | else
      |     set_param_state(gcb, 'exp_width', 'off')
      |     set_param_state(gcb, 'frac_width', 'off')
      | end
      mask Callback pipeline_cmult_en:
      | pipeline_en = get_param(gcb, 'pipeline_cmult_en');
      | if strcmp(pipeline_en,'on')
      | 
      |     set_param_state(gcb, 'pipeline_latency', 'on')
      | else
      |     set_param_state(gcb, 'pipeline_latency', 'off')
      | end
      mask TypeOptions multiplier_implementation: behavioral HDL | standard core | embedded multiplier core
      mask DialogControl ParameterTabVar0 Prompt: basic
      mask DialogControl ParameterTabVar01 Prompt: latency
      mask DialogControl ParameterTabVar012 Prompt: implementation
  cmult1 : Subsystem  AncestorBlock=casper_library_multipliers/cmult  mask(cmult){n_bits_a=bw, bin_pt_a=bw-1, n_bits_b=bw, bin_pt_b=bw-1, n_bits_ab=bw+bw+1, bin_pt_ab=bw-1 + bw-1, quantization=Truncate, overflow=Wrap, conjugated=on, async=off, pipelined_enable=off, floating_point=off, float_type=single, exp_width=8, frac_width=24, in_latency=0, mult_latency=3, add_latency=1, conv_latency=0, pipeline_cmult_en=off, pipeline_latency=0, multiplier_implementation=behavioral HDL}
      mask prompts: n_bits_a "Number of Bits 'a'"; bin_pt_a "Binary Point 'a'"; n_bits_b "Number of Bits 'b'"; bin_pt_b "Binary Point 'b'"; n_bits_ab "Number of Bits 'ab'"; bin_pt_ab "Binary Point 'ab'"; conjugated "Conjugate"; async "asynchronous operation"; pipelined_enable "enable pipeline"; floating_point "floating point"; float_type "float type"; exp_width "exponent width"; frac_width "fraction width"; in_latency "Input latency"; mult_latency "Multiplier Latency"; add_latency "Adder Latency"; conv_latency "Convert latency"; pipeline_cmult_en "Pipeline cmult enable"; pipeline_latency "Pipeline latency"; multiplier_implementation "Multiplier implementation"
      mask help:
      | Multiplies two complex numbers using 4 multipliers and 2 adders.
      | Conjugation is optional.
      mask init: same as snap_adc5g_spec/crosspower_vacc/cmult
      settings: AttributesFormatString=|
      | 18_17 * 18_17 ==> 37_34
      | Truncate, Wrap
      | Latency=0
      mask TypeOptions quantization: Truncate | Round  (unbiased: +/- Inf) | Round  (unbiased: Even Values)
      mask TypeOptions overflow: Wrap | Saturate | Flag as error
      mask Callback floating_point:
      | onoff = get_param(gcb, 'floating_point');
      | if strcmp(onoff,'on')
      |     enable_fixpt = 'off'
      |     set_param_state(gcb, 'float_type', 'on')
      | 
      |     f_type = get_param(gcb, 'float_type')
      |     if strcmp(f_type,'custom')
      |         set_param_state(gcb, 'exp_width', 'on')
      |         set_param_state(gcb, 'frac_width', 'on')
      |     else
      |         set_param_state(gcb, 'exp_width', 'off')
      |         set_param_state(gcb, 'frac_width', 'off')
      |     end
      | 
      | 
      | else
      |     enable_fixpt = 'on'
      |     set_param_state(gcb, 'float_type', 'off')
      |     set_param_state(gcb, 'exp_width', 'off')
      |     set_param_state(gcb, 'frac_width', 'off')
      | end
      | 
      | 
      | set_param_state(gcb, 'n_bits_a', enable_fixpt)
      | set_param_state(gcb, 'bin_pt_a', enable_fixpt)
      | set_param_state(gcb, 'n_bits_b', enable_fixpt)
      | set_param_state(gcb, 'bin_pt_b', enable_fixpt)
      | set_param_state(gcb, 'n_bits_ab', enable_fixpt)
      | set_param_state(gcb, 'bin_pt_ab', enable_fixpt)
      mask TypeOptions float_type: single | custom
      mask Callback float_type:
      | f_type = get_param(gcb, 'float_type')
      | if strcmp(f_type,'custom')
      |     set_param_state(gcb, 'exp_width', 'on')
      |     set_param_state(gcb, 'frac_width', 'on')
      | else
      |     set_param_state(gcb, 'exp_width', 'off')
      |     set_param_state(gcb, 'frac_width', 'off')
      | end
      mask Callback pipeline_cmult_en:
      | pipeline_en = get_param(gcb, 'pipeline_cmult_en');
      | if strcmp(pipeline_en,'on')
      | 
      |     set_param_state(gcb, 'pipeline_latency', 'on')
      | else
      |     set_param_state(gcb, 'pipeline_latency', 'off')
      | end
      mask TypeOptions multiplier_implementation: behavioral HDL | standard core | embedded multiplier core
      mask DialogControl ParameterTabVar0 Prompt: basic
      mask DialogControl ParameterTabVar01 Prompt: latency
      mask DialogControl ParameterTabVar012 Prompt: implementation
  detect_of : Subsystem
  detect_of1 : Subsystem
  detect_of2 : Subsystem
  detect_of3 : Subsystem
  of_count : Subsystem  Tag=xps:sw_reg  AncestorBlock=xps_library/Memory/software_register  mask(swreg){io_dir=To Processor, io_delay=0, init_val=0, sample_period=1, names=reg, bitwidths=32, bin_pts=0, arith_types=0, sim_port=on, show_format=on}
      mask prompts: io_dir "I/O direction"; io_delay "I/O delay"; init_val "Initial Value"; sample_period "Sample period"; names "Bitfield names [msb...lsb]"; bitwidths "Bitfield widths"; bin_pts "Bitfield binary pts"; arith_types "Bitfield types, ufix=0, fix=1, bool=2"; sim_port "Provide sim input/output?"; show_format "Print format string?"
      mask help: A 32-bit software-accessible register. Can be divided into bitfields of varying widths and types using the fields in the block mask.
      mask init:
      | swreg_init(gcb)
      settings: AttributesFormatString=1output:uf32.0 = 32 bits
      mask TypeOptions io_dir: To Processor | From Processor
      mask Callback io_dir:
      | mask_enables = get_param(gcb, 'MaskEnables');
      | mask_names = get_param(gcb, 'MaskNames');
      | if strcmp(get_param(gcb, 'io_dir'), 'To Processor'),
      |     mask_enables{ismember(mask_names, 'sample_period')} = 'off';
      | else
      |     mask_enables{ismember(mask_names, 'sample_period')} = 'on';
      | end
      | set_param(gcb, 'MaskEnables', mask_enables);
      mask DialogControl ParameterTabVar0 Prompt: Setup
  ri_to_c : casper_library_misc/ri_to_c
      settings: SourceProductName=CASPER DSP Blockset
  ri_to_c1 : casper_library_misc/ri_to_c
      settings: SourceProductName=CASPER DSP Blockset
  simple_bram_vacc : Subsystem  AncestorBlock=casper_library_accumulators/simple_bram_vacc  mask(simple_bram_vacc){vec_len=nchan/2, arith_type=Signed, n_bits=vacc_bw, bin_pt=vacc_bp}
      mask prompts: vec_len "Vector length:"; arith_type "Output type:"; n_bits "Bit width (output):"; bin_pt "Binary point (output):"
      mask help: This simple vector accumulator is based on a shift register. It outputs its previous accumulated vector after a new_acc pulse is received.
      mask init:
      | simple_bram_vacc_init(gcb, ...
      |     'vec_len', vec_len, ...
      |     'arith_type', arith_type, ...
      |     'n_bits', n_bits, ...
      |     'bin_pt', bin_pt);
      mask TypeOptions arith_type: Signed | Unsigned
  simple_bram_vacc1 : Subsystem  AncestorBlock=casper_library_accumulators/simple_bram_vacc  mask(simple_bram_vacc){vec_len=nchan/2, arith_type=Signed, n_bits=vacc_bw, bin_pt=vacc_bp}
      mask prompts: vec_len "Vector length:"; arith_type "Output type:"; n_bits "Bit width (output):"; bin_pt "Binary point (output):"
      mask help: This simple vector accumulator is based on a shift register. It outputs its previous accumulated vector after a new_acc pulse is received.
      mask init:
      | simple_bram_vacc_init(gcb, ...
      |     'vec_len', vec_len, ...
      |     'arith_type', arith_type, ...
      |     'n_bits', n_bits, ...
      |     'bin_pt', bin_pt);
      mask TypeOptions arith_type: Signed | Unsigned
  simple_bram_vacc2 : Subsystem  AncestorBlock=casper_library_accumulators/simple_bram_vacc  mask(simple_bram_vacc){vec_len=nchan/2, arith_type=Signed, n_bits=vacc_bw, bin_pt=vacc_bp}
      mask prompts: vec_len "Vector length:"; arith_type "Output type:"; n_bits "Bit width (output):"; bin_pt "Binary point (output):"
      mask help: This simple vector accumulator is based on a shift register. It outputs its previous accumulated vector after a new_acc pulse is received.
      mask init:
      | simple_bram_vacc_init(gcb, ...
      |     'vec_len', vec_len, ...
      |     'arith_type', arith_type, ...
      |     'n_bits', n_bits, ...
      |     'bin_pt', bin_pt);
      mask TypeOptions arith_type: Signed | Unsigned
  simple_bram_vacc3 : Subsystem  AncestorBlock=casper_library_accumulators/simple_bram_vacc  mask(simple_bram_vacc){vec_len=nchan/2, arith_type=Signed, n_bits=vacc_bw, bin_pt=vacc_bp}
      mask prompts: vec_len "Vector length:"; arith_type "Output type:"; n_bits "Bit width (output):"; bin_pt "Binary point (output):"
      mask help: This simple vector accumulator is based on a shift register. It outputs its previous accumulated vector after a new_acc pulse is received.
      mask init:
      | simple_bram_vacc_init(gcb, ...
      |     'vec_len', vec_len, ...
      |     'arith_type', arith_type, ...
      |     'n_bits', n_bits, ...
      |     'bin_pt', bin_pt);
      mask TypeOptions arith_type: Signed | Unsigned
  vld : Outport
  xy0 : Outport  Port=2
  xy1 : Outport  Port=3
  wires:
  simple_bram_vacc/2(valid) -> vld/1
  x0/1 -> cmult/1(a)
  new_acc/1 -> Delay/1
  x1/1 -> cmult1/1(a)
  y1/1 -> cmult1/2(b)
  y0/1 -> cmult/2(b)
  c_to_ri/2 -> detect_of1/1(in), Convert1/1
  c_to_ri/1 -> detect_of/1(in), Convert3/1
  cmult/1(ab) -> c_to_ri/1
  c_to_ri1/2 -> detect_of3/1(in), Convert4/1
  c_to_ri1/1 -> detect_of2/1(in), Convert2/1
  cmult1/1(ab) -> c_to_ri1/1
  Delay/1 -> Delay1/1
  simple_bram_vacc/1(dout) -> ri_to_c/1
  simple_bram_vacc1/1(dout) -> ri_to_c/2
  ri_to_c/1 -> xy0/1
  simple_bram_vacc2/1(dout) -> ri_to_c1/1
  simple_bram_vacc3/1(dout) -> ri_to_c1/2
  ri_to_c1/1 -> xy1/1
  Register/1 -> of_count/1(out_reg)
  Counter/1 -> Register/1
  Convert2/1 -> simple_bram_vacc2/2(din)
  Convert4/1 -> simple_bram_vacc3/2(din)
  Convert1/1 -> simple_bram_vacc1/2(din)
  Convert3/1 -> simple_bram_vacc/2(din)
  detect_of2/1(of) -> Logical/3
  detect_of1/1(of) -> Logical/2
  detect_of/1(of) -> Logical/1
  detect_of3/1(of) -> Logical/4
  Logical/1 -> Counter/2
  Delay1/1 -> simple_bram_vacc1/1(new_acc), simple_bram_vacc2/1(new_acc), simple_bram_vacc3/1(new_acc), Counter/1, Register/2, simple_bram_vacc/1(new_acc)

== system snap_adc5g_spec/fft_of ==
  out_reg : Inport
  assert_reg : xbsIndex_r4/Assert  assert_type=on  type_source=Explicitly  gui_display_data_type=Boolean  arith_type=Boolean  n_bits=1  bin_pt=0  preci_type=Single  exp_width=8  frac_width=24  assert_rate=off  rate_source=Explicitly  period=1  output_port=on  block_type=assert
  cast_gw : xbsIndex_r4/Convert  gui_display_data_type=Fixed-point  arith_type=Unsigned  n_bits=32  bin_pt=0  float_type=Single  exp_bits=8  fraction_bits=24  quantization=Truncate  overflow=Wrap  en=off  latency=1  pipeline=off  dbl_ovrd=off  block_type=convert
  io_delay : xbsIndex_r4/Delay  rst=off  infoeditControl=Selection of Reset will increase slice count due to use of real FFs and instead of SRLs  en=off  latency=0  reg_retiming=on  dbl_ovrd=off  block_type=delay
  reint1 : xbsIndex_r4/Reinterpret  force_arith_type=on  arith_type=Unsigned  force_bin_pt=on  bin_pt=0  block_type=reinterpret
  sim_out : Terminator
  sim_out_reg_gw : xbsIndex_r4/Gateway Out  inherit_from_input=off  hdl_port=off  rows=1  columns=1  UseAsDAC=off  DACChannel='1'  interface=None  automatic_assignment=on  address_offset=hex2dec('00')  intf_name=''  intf_description=''  timing_constraint=None  locs_specified=off  LOCs={}  io_standard={}  block_type=gatewayout
  sim_out_reg_sim_delay : xbsIndex_r4/Delay  rst=off  infoeditControl=Selection of Reset will increase slice count due to use of real FFs and instead of SRLs  en=off  latency=1  reg_retiming=on  dbl_ovrd=off  block_type=delay
  snap_adc5g_spec_fft_of_user_data_in : xbsIndex_r4/Gateway Out  inherit_from_input=off  hdl_port=on  rows=1  columns=1  UseAsDAC=off  DACChannel='1'  interface=None  automatic_assignment=on  address_offset=hex2dec('00')  intf_name=''  intf_description=''  timing_constraint=None  locs_specified=off  LOCs={}  io_standard={}  block_type=gatewayout
  sim_out_reg : Outport
  wires:
  sim_out_reg_sim_delay/1 -> sim_out_reg_gw/1
  sim_out_reg_gw/1 -> sim_out_reg/1
  io_delay/1 -> cast_gw/1
  cast_gw/1 -> snap_adc5g_spec_fft_of_user_data_in/1
  snap_adc5g_spec_fft_of_user_data_in/1 -> sim_out/1
  out_reg/1 -> sim_out_reg_sim_delay/1, assert_reg/1
  assert_reg/1 -> reint1/1
  reint1/1 -> io_delay/1
